simulink model "FMS"  (R2018b)
settings: configuration reference "fms_config" (kept outside this file)
values from neighbouring files (symbols this model uses):
  FMS_EXPORT = Simulink.Parameter(FMS_EXPORT_VALUE)    [fms_model_init.m]
  FMS_PARAM = Simulink.Parameter(FMS_PARAM_VALUE)    [fms_model_init.m]
undefined symbols (not defined in the file or in its folder): actuator_cmd, ax_cmd, ay_cmd, az_cmd, cmd_mask, ControlMode, ctrl_mode, DiscIntNeverNeededParam, ext_state, FMS_Cmd, FMS_CONST, home, mode, p_cmd, phi_cmd, PilotMode, psi_rate_cmd, q_cmd, r_cmd, reset, state, status, theta_cmd, throttle_cmd, timestamp, u_cmd, v_cmd, VehicleState, VehicleStatus, VTOLState, w_cmd, wp_consume, wp_current
libraries: simulink x141, FMT_Model_Lib x120, hdlsllib x13
(part 3 of 12)

== system FMS/FMS Commander/Commander/Arm/MC_Mode/SubMode/Takeoff ==
  FMS_In : Inport
  Action Port : ActionPort  InitializeStates=reset  ActionType=case
      settings: CopyFcn=Stateflow.SLINSF.SimulinkMan.removeBlockPreDeleteFcn
  Bus Assignment1 : BusAssignment  AssignedSignals=status,state,ctrl_mode,psi_rate_cmd,u_cmd,v_cmd,w_cmd
  Climb Speed : Subsystem
  Constant : Constant  Value=0  OutDataTypeStr=Inherit: Inherit via back propagation
  Constant1 : Constant  Value=0  OutDataTypeStr=Bus: FMS_Out_Bus
  Constant2 : Constant  Value=ControlMode.POSCTL
  Constant3 : Constant  Value=VehicleState.Takeoff
  Constant5 : Constant  Value=VehicleStatus.Arm
  Data Type Conversion : DataTypeConversion
  Data Type Conversion1 : DataTypeConversion
  Data Type Conversion2 : DataTypeConversion
  Demux : Demux  Outputs=2
  Track Position : Subsystem
  FMS_Out : Outport
  wires:
  Constant5/1 -> Data Type Conversion/1
  Demux/2 -> Bus Assignment1/7
  Demux/1 -> Bus Assignment1/6
  Constant/1 -> Bus Assignment1/5
  Constant2/1 -> Data Type Conversion2/1
  Track Position/1(uv_cmd_mPs) -> Demux/1
  Constant1/1 -> Bus Assignment1/1
  FMS_In/1 -> Climb Speed/1(FMS_In), Track Position/1(FMS_In)
  Bus Assignment1/1 -> FMS_Out/1
  Data Type Conversion/1 -> Bus Assignment1/2
  Data Type Conversion1/1 -> Bus Assignment1/3
  Constant3/1 -> Data Type Conversion1/1
  Data Type Conversion2/1 -> Bus Assignment1/4
  Climb Speed/1(w_cmd_mPs) -> Bus Assignment1/8

== system FMS/FMS Commander/Commander/Arm/MC_Mode/SubMode/Unknown ==
  Action Port : ActionPort  InitializeStates=reset  ActionType=default
  Bus Assignment : BusAssignment  AssignedSignals=reset,status,state,actuator_cmd
  Constant : Constant  Value=0  OutDataTypeStr=Bus: FMS_Out_Bus
  Constant1 : Constant  Value=VehicleStatus.Disarm
  Constant2 : Constant  OutDataTypeStr=Inherit: Inherit via back propagation
  Constant3 : Constant  Value=[1000;1000;1000;1000]  VectorParams1D=off  OutDataTypeStr=Inherit: Inherit via back propagation
  Constant4 : Constant  Value=zeros(12,1)  OutDataTypeStr=Inherit: Inherit via back propagation
  Constant5 : Constant  Value=VehicleState.Disarm
  Data Type Conversion : DataTypeConversion
  Data Type Conversion1 : DataTypeConversion
  Mux : Mux  Inputs=2
  FMS_Out : Outport
  wires:
  Mux/1 -> Bus Assignment/5
  Constant4/1 -> Mux/2
  Constant3/1 -> Mux/1
  Constant1/1 -> Data Type Conversion/1
  Constant2/1 -> Bus Assignment/2
  Bus Assignment/1 -> FMS_Out/1
  Constant/1 -> Bus Assignment/1
  Constant5/1 -> Data Type Conversion1/1
  Data Type Conversion/1 -> Bus Assignment/3
  Data Type Conversion1/1 -> Bus Assignment/4

== system FMS/FMS Commander/Commander/Arm/BackwardTrans_Mode/Position Command/Controller/Brake Control ==
  Action Port : ActionPort  InitializeStates=reset  ActionType=case
  Brake Speed : Constant  Value=0  VectorParams1D=off  OutDataTypeStr=single
  ay_cmd_mPs2 : Outport
  wires:
  Brake Speed/1 -> ay_cmd_mPs2/1

== system FMS/FMS Commander/Commander/Arm/BackwardTrans_Mode/Position Command/Controller/Hold Control ==
  note: Use L1 only if vehicle fly forward
  FMS_In : Inport
  Action Port : ActionPort  InitializeStates=reset  ActionType=case
  Bus Selector1 : BusSelector  OutputSignals=INS_Out.vn,INS_Out.ve
  FMS_In1 : InportShadow
  Fly_Direction : Subsystem
  L1 : Constant  Value=FMS_PARAM.FW_L1  OutDataTypeStr=single
  L1_Reference_WP : Subsystem
  Lateral_Acceleration : Subsystem
  Mux : Mux  Inputs=2
  Path_Ray : Subsystem
  Switch : Switch  Criteria=u2 > Threshold
  Velocity_Controller : Subsystem
  ay_cmd_mPs2 : Outport
  wires:
  FMS_In/1 -> Path_Ray/1(FMS_In)
  Path_Ray/1(p_vehicle) -> Lateral_Acceleration/1(p_vehicle), L1_Reference_WP/1(c)
  Path_Ray/2(p_0) -> L1_Reference_WP/2(p_0)
  Path_Ray/3(n) -> L1_Reference_WP/3(n)
  L1/1 -> L1_Reference_WP/4(L1), Lateral_Acceleration/3(L1)
  FMS_In1/1 -> Fly_Direction/1(FMS_In), Velocity_Controller/1(FMS_In), Bus Selector1/1
  Bus Selector1/1 -> Mux/1  "<vn>"
  Bus Selector1/2 -> Mux/2  "<ve>"
  L1_Reference_WP/1(L1_WP) -> Lateral_Acceleration/2(L1_WP)
  Mux/1 -> Lateral_Acceleration/4(Vg)
  Lateral_Acceleration/1(ay_cmd_mPs2) -> Switch/1
  Fly_Direction/1(sign) -> Switch/2
  Velocity_Controller/1(ay_cmd_B_rad) -> Switch/3
  Switch/1 -> ay_cmd_mPs2/1

== system FMS/FMS Commander/Commander/Arm/BackwardTrans_Mode/Position Command/Controller/Move Control ==
  FMS_In : Inport
  Action Port : ActionPort  InitializeStates=reset  ActionType=case
  Bus Selector : BusSelector  OutputSignals=Pilot_Cmd.stick_roll
  DeadZone1 : Subsystem  mask{th=FMS_PARAM.ROLL_DZ}
      mask prompts: th "Threshold"
      mask Display: disp('Dead Zone')
  Gain6 : Gain  Gain=FMS_PARAM.FW_ACC_Y_LIM/2  OutDataTypeStr=single
  TD : Subsystem  Commented=on
  ay_cmd_mPs2 : Outport
  wires:
  DeadZone1/1(y) -> Gain6/1
  Bus Selector/1 -> DeadZone1/1(u)  "<stick_roll>"
  FMS_In/1 -> Bus Selector/1
  Gain6/1 -> ay_cmd_mPs2/1

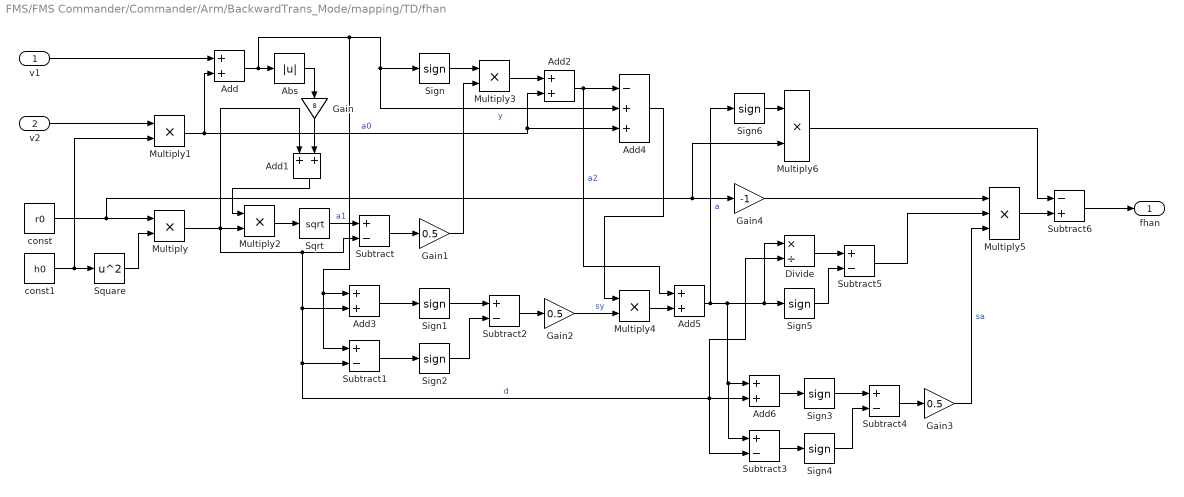
== system FMS/FMS Commander/Commander/Arm/BackwardTrans_Mode/mapping/TD/fhan  ==
  v1 : Inport
  v2 : Inport  Port=2
  Abs : Abs
  Add{,1..3,5..6} (6 alike) : Sum  OutDataTypeStr=Inherit: Same as first input
  Add4 : Sum  Inputs=-++
  Divide : Product  Inputs=*/
  Gain : Gain  Gain=8
  Gain1 : Gain  Gain=0.5  OutDataTypeStr=Inherit: Same as input
  Gain2 : Gain  Gain=0.5  OutDataTypeStr=Inherit: Same as input
  Gain3 : Gain  Gain=0.5  OutDataTypeStr=Inherit: Same as input
  Gain4 : Gain  Gain=-1  OutDataTypeStr=Inherit: Same as input
  Multiply{,1..3} (4 alike) : Product  OutDataTypeStr=Inherit: Same as first input
  Multiply4 : Product  OutDataTypeStr=single
  Multiply5 : Product  Inputs=3
  Multiply6 : Product  OutDataTypeStr=single
  Sign{,1..6} (7 alike) : Signum
  Sqrt : Sqrt  SaturateOnIntegerOverflow=on
  Square : Math  Operator=square  SaturateOnIntegerOverflow=on
  Subtract{,1..5} (6 alike) : Sum  Inputs=+-  OutDataTypeStr=Inherit: Same as first input
  Subtract6 : Sum  Inputs=-+  OutDataTypeStr=Inherit: Same as first input
  const : Constant  Value=r0  OutDataTypeStr=single
  const1 : Constant  Value=h0  OutDataTypeStr=single
  fhan : Outport
  wires:
  v1/1 -> Add/1
  Sign/1 -> Multiply3/1
  Gain2/1 -> Multiply4/2  "sy"
  v2/1 -> Multiply1/1
  Gain3/1 -> Multiply5/3  "sa"
  Subtract/1 -> Gain1/1
  Subtract6/1 -> fhan/1
  Sign2/1 -> Subtract2/2
  Sign4/1 -> Subtract4/2
  Abs/1 -> Gain/1
  Add4/1 -> Multiply4/1
  Sign5/1 -> Subtract5/2
  Sqrt/1 -> Subtract/1  "a1"
  Subtract3/1 -> Sign4/1
  Add1/1 -> Multiply2/1
  Subtract1/1 -> Sign2/1
  Divide/1 -> Subtract5/1
  Multiply3/1 -> Add2/1
  Gain/1 -> Add1/2
  const/1 -> Multiply6/2, Gain4/1, Multiply/1
  Add3/1 -> Sign1/1
  Subtract5/1 -> Multiply5/2
  Multiply4/1 -> Add5/2
  const1/1 -> Multiply1/2, Square/1
  Add5/1 -> Sign6/1, Sign5/1, Divide/1, Subtract3/1, Add6/1  "a"
  Multiply1/1 -> Add4/3, Add2/2, Add/2  "a0"
  Add/1 -> Subtract1/1, Add3/1, Add4/2, Sign/1, Abs/1  "y"
  Subtract2/1 -> Gain2/1
  Add2/1 -> Add4/1, Add5/1  "a2"
  Subtract4/1 -> Gain3/1
  Gain4/1 -> Multiply5/1
  Multiply5/1 -> Subtract6/2
  Sign6/1 -> Multiply6/1
  Sign3/1 -> Subtract4/1
  Add6/1 -> Sign3/1
  Multiply/1 -> Subtract/2, Divide/2, Subtract3/2, Add6/2, Subtract1/2, Add3/2, Add1/1, Multiply2/2  "d"
  Multiply6/1 -> Subtract6/1
  Gain1/1 -> Multiply3/2
  Square/1 -> Multiply/2
  Multiply2/1 -> Sqrt/1
  Sign1/1 -> Subtract2/1

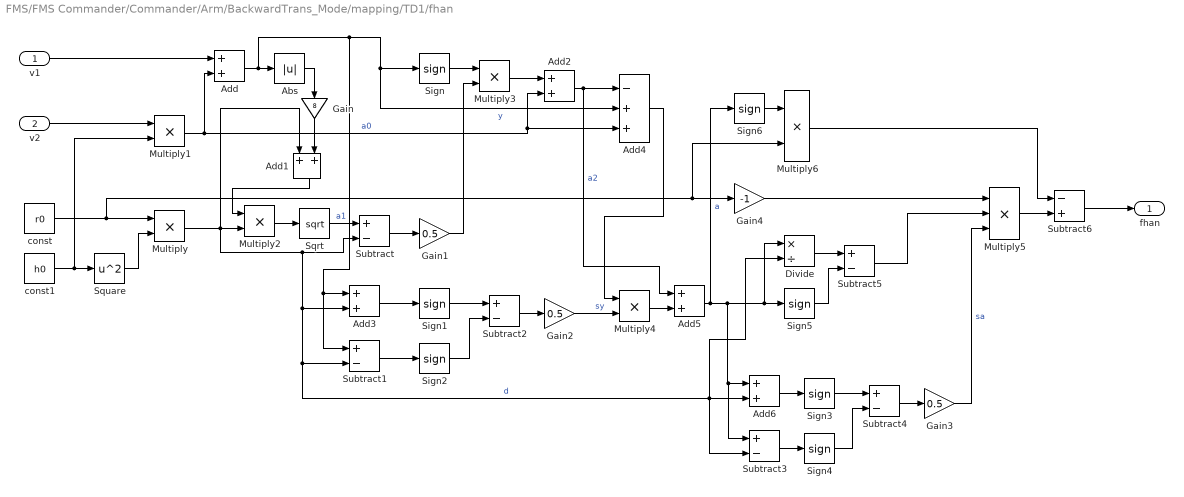
== system FMS/FMS Commander/Commander/Arm/BackwardTrans_Mode/mapping/TD1/fhan  ==
  v1 : Inport
  v2 : Inport  Port=2
  Abs : Abs
  Add{,1..3,5..6} (6 alike) : Sum  OutDataTypeStr=Inherit: Same as first input
  Add4 : Sum  Inputs=-++
  Divide : Product  Inputs=*/
  Gain : Gain  Gain=8
  Gain1 : Gain  Gain=0.5  OutDataTypeStr=Inherit: Same as input
  Gain2 : Gain  Gain=0.5  OutDataTypeStr=Inherit: Same as input
  Gain3 : Gain  Gain=0.5  OutDataTypeStr=Inherit: Same as input
  Gain4 : Gain  Gain=-1  OutDataTypeStr=Inherit: Same as input
  Multiply{,1..3} (4 alike) : Product  OutDataTypeStr=Inherit: Same as first input
  Multiply4 : Product  OutDataTypeStr=single
  Multiply5 : Product  Inputs=3
  Multiply6 : Product  OutDataTypeStr=single
  Sign{,1..6} (7 alike) : Signum
  Sqrt : Sqrt  SaturateOnIntegerOverflow=on
  Square : Math  Operator=square  SaturateOnIntegerOverflow=on
  Subtract{,1..5} (6 alike) : Sum  Inputs=+-  OutDataTypeStr=Inherit: Same as first input
  Subtract6 : Sum  Inputs=-+  OutDataTypeStr=Inherit: Same as first input
  const : Constant  Value=r0  OutDataTypeStr=single
  const1 : Constant  Value=h0  OutDataTypeStr=single
  fhan : Outport
  wires:
  v1/1 -> Add/1
  Sign/1 -> Multiply3/1
  Gain2/1 -> Multiply4/2  "sy"
  v2/1 -> Multiply1/1
  Gain3/1 -> Multiply5/3  "sa"
  Subtract/1 -> Gain1/1
  Subtract6/1 -> fhan/1
  Sign2/1 -> Subtract2/2
  Sign4/1 -> Subtract4/2
  Abs/1 -> Gain/1
  Add4/1 -> Multiply4/1
  Sign5/1 -> Subtract5/2
  Sqrt/1 -> Subtract/1  "a1"
  Subtract3/1 -> Sign4/1
  Add1/1 -> Multiply2/1
  Subtract1/1 -> Sign2/1
  Divide/1 -> Subtract5/1
  Multiply3/1 -> Add2/1
  Gain/1 -> Add1/2
  const/1 -> Multiply6/2, Gain4/1, Multiply/1
  Add3/1 -> Sign1/1
  Subtract5/1 -> Multiply5/2
  Multiply4/1 -> Add5/2
  const1/1 -> Multiply1/2, Square/1
  Add5/1 -> Sign6/1, Sign5/1, Divide/1, Subtract3/1, Add6/1  "a"
  Multiply1/1 -> Add4/3, Add2/2, Add/2  "a0"
  Add/1 -> Subtract1/1, Add3/1, Add4/2, Sign/1, Abs/1  "y"
  Subtract2/1 -> Gain2/1
  Add2/1 -> Add4/1, Add5/1  "a2"
  Subtract4/1 -> Gain3/1
  Gain4/1 -> Multiply5/1
  Multiply5/1 -> Subtract6/2
  Sign6/1 -> Multiply6/1
  Sign3/1 -> Subtract4/1
  Add6/1 -> Sign3/1
  Multiply/1 -> Subtract/2, Divide/2, Subtract3/2, Add6/2, Subtract1/2, Add3/2, Add1/1, Multiply2/2  "d"
  Multiply6/1 -> Subtract6/1
  Gain1/1 -> Multiply3/2
  Square/1 -> Multiply/2
  Multiply2/1 -> Sqrt/1
  Sign1/1 -> Subtract2/1

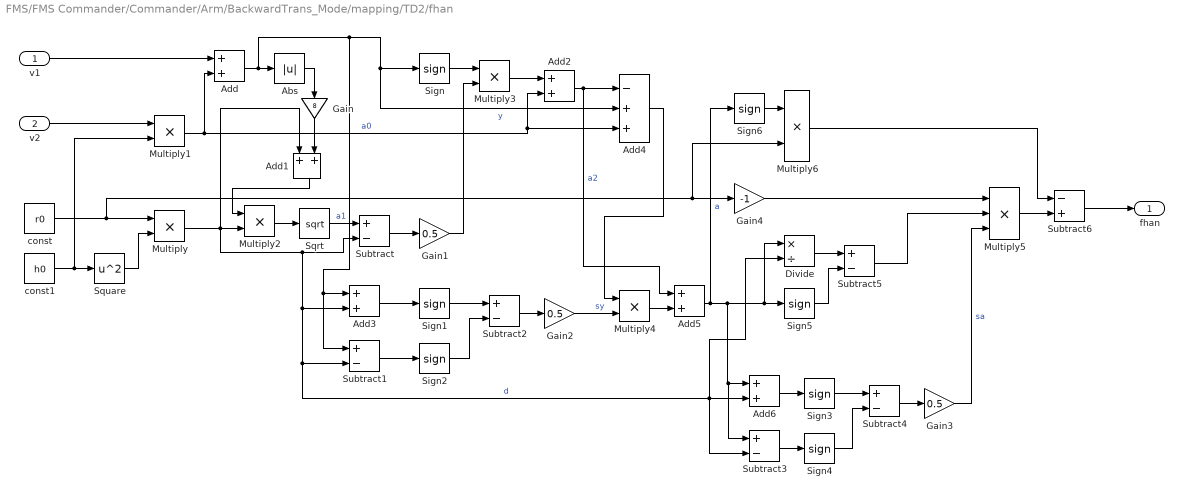
== system FMS/FMS Commander/Commander/Arm/BackwardTrans_Mode/mapping/TD2/fhan  ==
  v1 : Inport
  v2 : Inport  Port=2
  Abs : Abs
  Add{,1..3,5..6} (6 alike) : Sum  OutDataTypeStr=Inherit: Same as first input
  Add4 : Sum  Inputs=-++
  Divide : Product  Inputs=*/
  Gain : Gain  Gain=8
  Gain1 : Gain  Gain=0.5  OutDataTypeStr=Inherit: Same as input
  Gain2 : Gain  Gain=0.5  OutDataTypeStr=Inherit: Same as input
  Gain3 : Gain  Gain=0.5  OutDataTypeStr=Inherit: Same as input
  Gain4 : Gain  Gain=-1  OutDataTypeStr=Inherit: Same as input
  Multiply{,1..3} (4 alike) : Product  OutDataTypeStr=Inherit: Same as first input
  Multiply4 : Product  OutDataTypeStr=single
  Multiply5 : Product  Inputs=3
  Multiply6 : Product  OutDataTypeStr=single
  Sign{,1..6} (7 alike) : Signum
  Sqrt : Sqrt  SaturateOnIntegerOverflow=on
  Square : Math  Operator=square  SaturateOnIntegerOverflow=on
  Subtract{,1..5} (6 alike) : Sum  Inputs=+-  OutDataTypeStr=Inherit: Same as first input
  Subtract6 : Sum  Inputs=-+  OutDataTypeStr=Inherit: Same as first input
  const : Constant  Value=r0  OutDataTypeStr=single
  const1 : Constant  Value=h0  OutDataTypeStr=single
  fhan : Outport
  wires:
  Sign1/1 -> Subtract2/1
  Multiply2/1 -> Sqrt/1
  Square/1 -> Multiply/2
  Gain1/1 -> Multiply3/2
  Multiply6/1 -> Subtract6/1
  Multiply/1 -> Multiply2/2, Add1/1, Add3/2, Subtract1/2, Add6/2, Subtract3/2, Divide/2, Subtract/2  "d"
  Add6/1 -> Sign3/1
  Sign3/1 -> Subtract4/1
  Sign6/1 -> Multiply6/1
  Multiply5/1 -> Subtract6/2
  Gain4/1 -> Multiply5/1
  Subtract4/1 -> Gain3/1
  Add2/1 -> Add5/1, Add4/1  "a2"
  Subtract2/1 -> Gain2/1
  Add/1 -> Abs/1, Sign/1, Add4/2, Add3/1, Subtract1/1  "y"
  Multiply1/1 -> Add/2, Add2/2, Add4/3  "a0"
  Add5/1 -> Add6/1, Subtract3/1, Divide/1, Sign5/1, Sign6/1  "a"
  const1/1 -> Square/1, Multiply1/2
  Multiply4/1 -> Add5/2
  Subtract5/1 -> Multiply5/2
  Add3/1 -> Sign1/1
  const/1 -> Multiply/1, Gain4/1, Multiply6/2
  Gain/1 -> Add1/2
  Multiply3/1 -> Add2/1
  Divide/1 -> Subtract5/1
  Subtract1/1 -> Sign2/1
  Add1/1 -> Multiply2/1
  Subtract3/1 -> Sign4/1
  Sqrt/1 -> Subtract/1  "a1"
  Sign5/1 -> Subtract5/2
  Add4/1 -> Multiply4/1
  Abs/1 -> Gain/1
  Sign4/1 -> Subtract4/2
  Sign2/1 -> Subtract2/2
  Subtract6/1 -> fhan/1
  Subtract/1 -> Gain1/1
  Gain3/1 -> Multiply5/3  "sa"
  v2/1 -> Multiply1/1
  Gain2/1 -> Multiply4/2  "sy"
  Sign/1 -> Multiply3/1
  v1/1 -> Add/1

== system FMS/FMS Commander/Commander/Arm/FW_Mode/Assist/Altitude/Altitude Command ==
  FMS_In : Inport
  Controller : Subsystem
  Detect Movement : Subsystem
  w_cmd_mPs : Outport
  wires:
  Controller/1(w_cmd_mPs) -> w_cmd_mPs/1
  Detect Movement/1(motion_state) -> Controller/1(motion_state)
  FMS_In/1 -> Controller/2(FMS_In), Detect Movement/1(FMS_In)

== system FMS/FMS Commander/Commander/Arm/FW_Mode/Assist/Altitude/Attitude Command ==
  FMS_In : Inport
  Bus Selector : BusSelector  OutputSignals=Pilot_Cmd.stick_roll
  DeadZone : Subsystem  mask{th=FMS_PARAM.ROLL_DZ}
      mask prompts: th "Threshold"
      mask Display: disp('Dead Zone')
  Gain : Gain  Gain=FMS_PARAM.FW_ROLL_LIM
  TD : Subsystem
  phi_cmd_radPs : Outport
  wires:
  Bus Selector/1 -> DeadZone/1(u)  "<stick_roll>"
  FMS_In/1 -> Bus Selector/1
  DeadZone/1(y) -> Gain/1
  Gain/1 -> TD/1(v)
  TD/1(v1) -> phi_cmd_radPs/1

== system FMS/FMS Commander/Commander/Arm/FW_Mode/Assist/Altitude/Heading Command ==
  FMS_In : Inport
  Bus Selector : BusSelector  OutputSignals=Pilot_Cmd.stick_yaw
  DeadZone : Subsystem  mask{th=FMS_PARAM.YAW_DZ}
      mask prompts: th "Threshold"
      mask Display: disp('Dead Zone')
  Gain1 : Gain  Gain=FMS_PARAM.FW_YAW_RATE_LIM  OutDataTypeStr=single
  TD : Subsystem
  psi_rate_cmd_radPs : Outport
  wires:
  Gain1/1 -> TD/1(v)
  FMS_In/1 -> Bus Selector/1
  DeadZone/1(y) -> Gain1/1
  Bus Selector/1 -> DeadZone/1(u)  "<stick_yaw>"
  TD/1(v1) -> psi_rate_cmd_radPs/1

== system FMS/FMS Commander/Commander/Arm/FW_Mode/Assist/Altitude/Speed Command ==
  FMS_In : Inport
  Bus Selector : BusSelector  OutputSignals=Pilot_Cmd.stick_throttle
  Saturation : Saturate  UpperLimit=1  LowerLimit=-1
  Saturation1 : Saturate  UpperLimit=FMS_PARAM.FW_SPEED_MAX  LowerLimit=FMS_PARAM.FW_SPEED_MIN
  StickToVelMapping : Subsystem  mask{min=FMS_PARAM.FW_SPEED_MIN, mid=FMS_PARAM.FW_CRUISE_SPEED, max=FMS_PARAM.FW_SPEED_MAX}
  TD : Subsystem
  u_cmd_mPs : Outport
  wires:
  FMS_In/1 -> Bus Selector/1
  Bus Selector/1 -> Saturation/1  "<stick_throttle>"
  Saturation/1 -> StickToVelMapping/1(In)
  StickToVelMapping/1(Out) -> TD/1(v)
  Saturation1/1 -> u_cmd_mPs/1
  TD/1(v1) -> Saturation1/1

== system FMS/FMS Commander/Commander/Arm/FW_Mode/Assist/Position/Altitude Command ==
  FMS_In : Inport
  Controller : Subsystem
  Detect Movement : Subsystem
  w_cmd_mPs : Outport
  wires:
  Controller/1(w_cmd_mPs) -> w_cmd_mPs/1
  Detect Movement/1(motion_state) -> Controller/1(motion_state)
  FMS_In/1 -> Controller/2(FMS_In), Detect Movement/1(FMS_In)

== system FMS/FMS Commander/Commander/Arm/FW_Mode/Assist/Position/Heading Command ==
  FMS_In : Inport
  Bus Selector : BusSelector  OutputSignals=Pilot_Cmd.stick_yaw
  DeadZone : Subsystem  mask{th=FMS_PARAM.YAW_DZ}
      mask prompts: th "Threshold"
      mask Display: disp('Dead Zone')
  Gain1 : Gain  Gain=FMS_PARAM.FW_YAW_RATE_LIM  OutDataTypeStr=single
  TD : Subsystem
  psi_rate_cmd_radPs : Outport
  wires:
  Gain1/1 -> TD/1(v)
  FMS_In/1 -> Bus Selector/1
  DeadZone/1(y) -> Gain1/1
  Bus Selector/1 -> DeadZone/1(u)  "<stick_yaw>"
  TD/1(v1) -> psi_rate_cmd_radPs/1

== system FMS/FMS Commander/Commander/Arm/FW_Mode/Assist/Position/Position Command ==
  FMS_In : Inport
  Controller : Subsystem
  Detect Movement : Subsystem
  ay_cmd_mPs2 : Outport
  wires:
  FMS_In/1 -> Controller/2(FMS_In), Detect Movement/1(FMS_In)
  Controller/1(ay_cmd_mPs2) -> ay_cmd_mPs2/1
  Detect Movement/1(motion_state) -> Controller/1(motion_state)

== system FMS/FMS Commander/Commander/Arm/FW_Mode/Assist/Position/Speed Command ==
  FMS_In : Inport
  Bus Selector : BusSelector  OutputSignals=Pilot_Cmd.stick_throttle
  Saturation : Saturate  UpperLimit=1  LowerLimit=-1
  Saturation1 : Saturate  UpperLimit=FMS_PARAM.FW_SPEED_MAX  LowerLimit=FMS_PARAM.FW_SPEED_MIN
  StickToVelMapping : Subsystem  mask{min=FMS_PARAM.FW_SPEED_MIN, mid=FMS_PARAM.FW_CRUISE_SPEED, max=FMS_PARAM.FW_SPEED_MAX}
  TD : Subsystem
  u_cmd_mPs : Outport
  wires:
  FMS_In/1 -> Bus Selector/1
  Bus Selector/1 -> Saturation/1  "<stick_throttle>"
  Saturation/1 -> StickToVelMapping/1(In)
  StickToVelMapping/1(Out) -> TD/1(v)
  Saturation1/1 -> u_cmd_mPs/1
  TD/1(v1) -> Saturation1/1

== system FMS/FMS Commander/Commander/Arm/FW_Mode/Assist/Stabilize/Attitude Command ==
  FMS_In : Inport
  Bus Selector : BusSelector  OutputSignals=Pilot_Cmd.stick_roll,Pilot_Cmd.stick_pitch
  DeadZone : Subsystem  mask{th=FMS_PARAM.ROLL_DZ}
      mask prompts: th "Threshold"
      mask Display: disp('Dead Zone')
  DeadZone2 : Subsystem  mask{th=FMS_PARAM.PITCH_DZ}
      mask prompts: th "Threshold"
      mask Display: disp('Dead Zone')
  Gain : Gain  Gain=FMS_PARAM.FW_ROLL_LIM
  Gain1 : Gain  Gain=-FMS_PARAM.FW_PITCH_LIM
  Phi_CMD_TD : Subsystem
  Theta_CMD_TD : Subsystem
  phi_cmd_radPs : Outport
  theta_cmd_radPs : Outport  Port=2
  wires:
  Bus Selector/2 -> DeadZone2/1(u)  "<stick_pitch>"
  Bus Selector/1 -> DeadZone/1(u)  "<stick_roll>"
  FMS_In/1 -> Bus Selector/1
  DeadZone2/1(y) -> Gain1/1
  DeadZone/1(y) -> Gain/1
  Gain/1 -> Phi_CMD_TD/1(v)
  Gain1/1 -> Theta_CMD_TD/1(v)
  Phi_CMD_TD/1(v1) -> phi_cmd_radPs/1
  Theta_CMD_TD/1(v1) -> theta_cmd_radPs/1

== system FMS/FMS Commander/Commander/Arm/FW_Mode/Assist/Stabilize/Heading Command ==
  FMS_In : Inport
  Bus Selector : BusSelector  OutputSignals=Pilot_Cmd.stick_yaw
  DeadZone : Subsystem  mask{th=FMS_PARAM.YAW_DZ}
      mask prompts: th "Threshold"
      mask Display: disp('Dead Zone')
  Gain1 : Gain  Gain=FMS_PARAM.FW_YAW_RATE_LIM  OutDataTypeStr=single
  TD : Subsystem
  psi_rate_cmd_radPs : Outport
  wires:
  Gain1/1 -> TD/1(v)
  FMS_In/1 -> Bus Selector/1
  DeadZone/1(y) -> Gain1/1
  Bus Selector/1 -> DeadZone/1(u)  "<stick_yaw>"
  TD/1(v1) -> psi_rate_cmd_radPs/1

== system FMS/FMS Commander/Commander/Arm/FW_Mode/Assist/Stabilize/Throttle Command ==
  FMS_In : Inport
  Add : Sum
  Bus Selector : BusSelector  OutputSignals=Pilot_Cmd.stick_throttle
  Constant5 : Constant  Value=1000  OutDataTypeStr=uint16
  Gain2 : Gain  Gain=1000  OutDataTypeStr=uint16
  Saturation : Saturate  UpperLimit=1  LowerLimit=0
  throttle_cmd : Outport
  wires:
  FMS_In/1 -> Bus Selector/1
  Gain2/1 -> Add/1
  Saturation/1 -> Gain2/1
  Bus Selector/1 -> Saturation/1  "<stick_throttle>"
  Constant5/1 -> Add/2
  Add/1 -> throttle_cmd/1

== system FMS/FMS Commander/Commander/Arm/FW_Mode/Auto/Mission/Mission_SubSystem ==
  FMS_In : Inport
  Reset : ResetPort  DisableCoverage=on
  Altitude Control : Subsystem
  Bus Assignment : BusAssignment  AssignedSignals=status,state,ctrl_mode,u_cmd,ay_cmd,w_cmd
  Constant : Constant  Value=0  OutDataTypeStr=Bus: FMS_Out_Bus
  Constant1 : Constant  Value=VehicleStatus.Arm
  Constant2 : Constant  Value=VehicleState.Mission
  Constant3 : Constant  Value=ControlMode.POSCTL
  Cruise_Speed : Subsystem
  Data Type Conversion : DataTypeConversion
  Data Type Conversion1 : DataTypeConversion
  Data Type Conversion2 : DataTypeConversion
  Position Command : Subsystem
  FMS_Out : Outport
  wires:
  Data Type Conversion1/1 -> Bus Assignment/3
  Constant1/1 -> Data Type Conversion/1
  Data Type Conversion2/1 -> Bus Assignment/4
  Data Type Conversion/1 -> Bus Assignment/2
  Constant2/1 -> Data Type Conversion1/1
  Constant3/1 -> Data Type Conversion2/1
  Constant/1 -> Bus Assignment/1
  Bus Assignment/1 -> FMS_Out/1
  FMS_In/1 -> Cruise_Speed/1(FMS_In), Altitude Control/1(FMS_In), Position Command/1(FMS_In)
  Position Command/1(ay_cmd_mPs2) -> Bus Assignment/6
  Altitude Control/1(w_cmd_mPs) -> Bus Assignment/7
  Cruise_Speed/1(u_cmd) -> Bus Assignment/5

== system FMS/FMS Commander/Commander/Arm/FW_Mode/SubMode/Hold/Altitude_Hold ==
  FMS_In : Inport
  Bus_Selection : Subsystem
  Delay : Delay  DelayLength=1  InitialConditionSource=Input port
      settings: InputPortMap=u0,p4
  Gain2 : Gain  Gain=FMS_PARAM.Z_P  OutDataTypeStr=single
  Saturation1 : Saturate  UpperLimit=FMS_PARAM.VEL_Z_LIM  LowerLimit=-FMS_PARAM.VEL_Z_LIM
  Sum : Sum  Inputs=-+|
  w_cmd_mPs : Outport
  wires:
  Gain2/1 -> Saturation1/1
  Bus_Selection/1(z_R_m) -> Delay/2, Sum/1  "z_est_R"
  Sum/1 -> Gain2/1  "z_err_R"
  Delay/1 -> Sum/2, Delay/1  "z_cmd_R"
  FMS_In/1 -> Bus_Selection/1(FMS_In)
  Saturation1/1 -> w_cmd_mPs/1

== system FMS/FMS Commander/Commander/Arm/FW_Mode/SubMode/Hold/Loiter_Control ==
  FMS_In : Inport
  Bus Selector2 : BusSelector  OutputSignals=INS_Out.vn,INS_Out.ve
  L1 : Constant  Value=FMS_PARAM.FW_L1  OutDataTypeStr=single
  L1 Reference WP : Subsystem
  L1_Core : Subsystem
  Mux1 : Mux  Inputs=2
  R : Constant  Value=FMS_PARAM.FW_LOITER_R  OutDataTypeStr=single
  Reference_Point : Subsystem
  Saturation1 : Saturate  UpperLimit=FMS_PARAM.FW_ACC_Y_LIM  LowerLimit=-FMS_PARAM.FW_ACC_Y_LIM
  ay_cmd_mPs2 : Outport
  wires:
  L1 Reference WP/1(L1_WP) -> L1_Core/2(L1_WP)  "L1_WP"
  L1_Core/1(ay_cmd_mPs2) -> Saturation1/1
  Reference_Point/1(p_vehicle) -> L1_Core/1(p_vehicle), L1 Reference WP/1(P_Vehicle)
  Reference_Point/2(p_0) -> L1 Reference WP/2(P_0)
  Reference_Point/3(n) -> L1 Reference WP/3(n)
  R/1 -> L1 Reference WP/4(R)
  L1/1 -> L1_Core/3(L1), L1 Reference WP/5(L1)
  FMS_In/1 -> Bus Selector2/1, Reference_Point/1(FMS_In)
  Bus Selector2/2 -> Mux1/2  "<ve>"
  Bus Selector2/1 -> Mux1/1  "<vn>"
  Mux1/1 -> L1_Core/4(Vg)
  Saturation1/1 -> ay_cmd_mPs2/1

== system FMS/FMS Commander/Commander/Arm/FW_Mode/SubMode/Return/Altitude Control ==
  FMS_In : Inport
  Bus Selector3 : BusSelector  OutputSignals=INS_Out.h_R
  Gain : Gain  Gain=FMS_PARAM.FW_Z_P
  Saturation1 : Saturate  UpperLimit=FMS_PARAM.FW_VEL_Z_LIM  LowerLimit=-FMS_PARAM.FW_VEL_Z_LIM
  Sum2 : Sum  Inputs=|+-
  Target Height : Subsystem
  w_cmd_mPs : Outport
  wires:
  FMS_In/1 -> Bus Selector3/1, Target Height/1(FMS_In)
  Bus Selector3/1 -> Sum2/1  "<h_R>"
  Sum2/1 -> Gain/1
  Gain/1 -> Saturation1/1
  Target Height/1(h_R_sp) -> Sum2/2  "h_R_sp"
  Saturation1/1 -> w_cmd_mPs/1

== system FMS/FMS Commander/Commander/Arm/FW_Mode/SubMode/Return/Position Command ==
  FMS_In : Inport
  L1 Control : Subsystem
  WayPoints : Subsystem
  ay_cmd_mPs2 : Outport
  wires:
  FMS_In/1 -> L1 Control/4(FMS_In), WayPoints/1(FMS_In)
  L1 Control/1(ay_cmd_mPs2) -> ay_cmd_mPs2/1
  WayPoints/2(p2) -> L1 Control/2(p2)
  WayPoints/3(p3) -> L1 Control/3(p3)
  WayPoints/1(p1) -> L1 Control/1(p1)

== system FMS/FMS Commander/Commander/Arm/FW_Mode/SubMode/Takeoff/Altitude Control ==
  FMS_In : Inport
  Bus Selector3 : BusSelector  OutputSignals=INS_Out.h_R
  Gain : Gain  Gain=FMS_PARAM.FW_Z_P
  Saturation1 : Saturate  UpperLimit=FMS_PARAM.FW_VEL_Z_LIM  LowerLimit=-FMS_PARAM.FW_VEL_Z_LIM
  Sum2 : Sum  Inputs=|+-
  Target Height : Subsystem
  w_cmd_mPs : Outport
  wires:
  FMS_In/1 -> Bus Selector3/1, Target Height/1(FMS_In)
  Bus Selector3/1 -> Sum2/1  "<h_R>"
  Sum2/1 -> Gain/1
  Gain/1 -> Saturation1/1
  Target Height/1(h_R_sp) -> Sum2/2  "h_R_sp"
  Saturation1/1 -> w_cmd_mPs/1

== system FMS/FMS Commander/Commander/Arm/FW_Mode/SubMode/Takeoff/Position Command ==
  FMS_In : Inport
  L1 Control : Subsystem
  WayPoints : Subsystem
  ay_cmd_mPs2 : Outport
  wires:
  FMS_In/1 -> L1 Control/4(FMS_In), WayPoints/1(FMS_In)
  L1 Control/1(ay_cmd_mPs2) -> ay_cmd_mPs2/1
  WayPoints/2(p2) -> L1 Control/2(p2)
  WayPoints/3(p3) -> L1 Control/3(p3)
  WayPoints/1(p1) -> L1 Control/1(p1)

== system FMS/FMS Commander/Commander/Arm/MC_Mode/Assist/Acro/Angular Rate Command ==
  FMS_In : Inport
  Bus Selector : BusSelector  OutputSignals=Pilot_Cmd.stick_roll,Pilot_Cmd.stick_pitch,Pilot_Cmd.stick_yaw
  Gain : Gain  Gain=pi  OutDataTypeStr=single
  Gain1 : Gain  Gain=-pi  OutDataTypeStr=single
  Gain2 : Gain  Gain=pi/2  OutDataTypeStr=single
  p_cmd_radPs : Outport
  q_cmd_radPs : Outport  Port=2
  r_cmd_radPs : Outport  Port=3
  wires:
  FMS_In/1 -> Bus Selector/1
  Gain2/1 -> r_cmd_radPs/1
  Gain1/1 -> q_cmd_radPs/1
  Bus Selector/3 -> Gain2/1  "<stick_yaw>"
  Bus Selector/2 -> Gain1/1  "<stick_pitch>"
  Gain/1 -> p_cmd_radPs/1
  Bus Selector/1 -> Gain/1  "<stick_roll>"

== system FMS/FMS Commander/Commander/Arm/MC_Mode/Assist/Acro/Throttle Command ==
  FMS_In : Inport
  Add : Sum
  Bus Selector : BusSelector  OutputSignals=Pilot_Cmd.stick_throttle
  Constant4 : Constant  OutDataTypeStr=single
  Constant5 : Constant  Value=1000  OutDataTypeStr=uint16
  Gain2 : Gain  Gain=500  OutDataTypeStr=uint16
  Saturation : Saturate  UpperLimit=2  LowerLimit=0
  Sum : Sum  Inputs=|++
  throttle_cmd : Outport
  wires:
  Constant4/1 -> Sum/2
  Add/1 -> throttle_cmd/1
  Constant5/1 -> Add/2
  Bus Selector/1 -> Sum/1  "<stick_throttle>"
  Saturation/1 -> Gain2/1
  Sum/1 -> Saturation/1
  Gain2/1 -> Add/1
  FMS_In/1 -> Bus Selector/1

== system FMS/FMS Commander/Commander/Arm/MC_Mode/Assist/Altitude/Altitude Command ==
  FMS_In : Inport
  Bus Selector : BusSelector  OutputSignals=pilot_cmd_lost
  Constant : Constant  Value=0.5  OutDataTypeStr=single
  Controller : Subsystem
  Detect Movement : Subsystem
  Switch : Switch  Criteria=u2 > Threshold
  w_cmd_mPs : Outport
  wires:
  Controller/1(w_cmd_mPs) -> Switch/3
  Detect Movement/1(motion_state) -> Controller/1(motion_state)
  FMS_In/1 -> Bus Selector/1, Controller/2(FMS_In), Detect Movement/1(FMS_In)
  Bus Selector/1 -> Switch/2  "<pilot_cmd_lost>"
  Constant/1 -> Switch/1
  Switch/1 -> w_cmd_mPs/1

== system FMS/FMS Commander/Commander/Arm/MC_Mode/Assist/Altitude/Attitude Command ==
  FMS_In : Inport
  Bus Selector : BusSelector  OutputSignals=Pilot_Cmd.stick_roll,Pilot_Cmd.stick_pitch
  Bus Selector1 : BusSelector  OutputSignals=pilot_cmd_lost
  Data Type Conversion : DataTypeConversion  OutDataTypeStr=single
  DeadZone : Subsystem  mask{th=FMS_PARAM.ROLL_DZ}
      mask prompts: th "Threshold"
      mask Display: disp('Dead Zone')
  DeadZone2 : Subsystem  mask{th=FMS_PARAM.PITCH_DZ}
      mask prompts: th "Threshold"
      mask Display: disp('Dead Zone')
  Gain : Gain  Gain=FMS_PARAM.ROLL_PITCH_LIM
  Gain1 : Gain  Gain=-FMS_PARAM.ROLL_PITCH_LIM
  Logical Operator : Logic  Operator=NOT  AllPortsSameDT=off  OutDataTypeStr=boolean
  Multiply : Product
  Multiply1 : Product
  Phi_CMD_TD : Subsystem
  Theta_CMD_TD : Subsystem
  phi_cmd_radPs : Outport
  theta_cmd_radPs : Outport  Port=2
  wires:
  Bus Selector/2 -> DeadZone2/1(u)  "<stick_pitch>"
  Bus Selector/1 -> DeadZone/1(u)  "<stick_roll>"
  FMS_In/1 -> Bus Selector1/1, Bus Selector/1
  Phi_CMD_TD/1(v1) -> Multiply/2
  Gain1/1 -> Theta_CMD_TD/1(v)
  Gain/1 -> Phi_CMD_TD/1(v)
  DeadZone2/1(y) -> Gain1/1
  DeadZone/1(y) -> Gain/1
  Bus Selector1/1 -> Logical Operator/1  "<pilot_cmd_lost>"
  Multiply/1 -> phi_cmd_radPs/1
  Theta_CMD_TD/1(v1) -> Multiply1/2
  Multiply1/1 -> theta_cmd_radPs/1
  Logical Operator/1 -> Data Type Conversion/1
  Data Type Conversion/1 -> Multiply1/1, Multiply/1

== system FMS/FMS Commander/Commander/Arm/MC_Mode/Assist/Altitude/Heading Command ==
  FMS_In : Inport
  Controller : Subsystem
  Detect Movement : Subsystem
  psi_rate_cmd_radPs : Outport
  wires:
  Controller/1(psi_rate_cmd_radPs) -> psi_rate_cmd_radPs/1
  Detect Movement/1(motion_state) -> Controller/1(motion_state)
  FMS_In/1 -> Controller/2(FMS_In), Detect Movement/1(FMS_In)

== system FMS/FMS Commander/Commander/Arm/MC_Mode/Assist/Position/Altitude Command ==
  FMS_In : Inport
  Controller : Subsystem
  Detect Movement : Subsystem
  w_cmd_mPs : Outport
  wires:
  Controller/1(w_cmd_mPs) -> w_cmd_mPs/1
  Detect Movement/1(motion_state) -> Controller/1(motion_state)
  FMS_In/1 -> Controller/2(FMS_In), Detect Movement/1(FMS_In)

== system FMS/FMS Commander/Commander/Arm/MC_Mode/Assist/Position/Heading Command ==
  FMS_In : Inport
  Controller : Subsystem
  Detect Movement : Subsystem
  psi_rate_cmd_radPs : Outport
  wires:
  Controller/1(psi_rate_cmd_radPs) -> psi_rate_cmd_radPs/1
  Detect Movement/1(motion_state) -> Controller/1(motion_state)
  FMS_In/1 -> Controller/2(FMS_In), Detect Movement/1(FMS_In)

== system FMS/FMS Commander/Commander/Arm/MC_Mode/Assist/Position/Position Command ==
  FMS_In : Inport
  Controller : Subsystem
  Demux : Demux  Outputs=2
  Detect Movement : Subsystem
  u_cmd_mPs : Outport
  v_cmd_mPs : Outport  Port=2
  wires:
  FMS_In/1 -> Controller/2(FMS_In), Detect Movement/1(FMS_In)
  Demux/2 -> v_cmd_mPs/1
  Demux/1 -> u_cmd_mPs/1
  Controller/1(uv_cmd_mPs) -> Demux/1
  Detect Movement/1(motion_state) -> Controller/1(motion_state)

== system FMS/FMS Commander/Commander/Arm/MC_Mode/Assist/Stabilize/Attitude Command ==
  FMS_In : Inport
  Bus Selector : BusSelector  OutputSignals=Pilot_Cmd.stick_roll,Pilot_Cmd.stick_pitch
  Bus Selector1 : BusSelector  OutputSignals=pilot_cmd_lost
  Data Type Conversion : DataTypeConversion  OutDataTypeStr=single
  DeadZone : Subsystem  mask{th=FMS_PARAM.ROLL_DZ}
      mask prompts: th "Threshold"
      mask Display: disp('Dead Zone')
  DeadZone2 : Subsystem  mask{th=FMS_PARAM.PITCH_DZ}
      mask prompts: th "Threshold"
      mask Display: disp('Dead Zone')
  Gain : Gain  Gain=FMS_PARAM.ROLL_PITCH_LIM
  Gain1 : Gain  Gain=-FMS_PARAM.ROLL_PITCH_LIM
  Logical Operator : Logic  Operator=NOT  AllPortsSameDT=off  OutDataTypeStr=boolean
  Multiply : Product
  Multiply1 : Product
  Phi_CMD_TD : Subsystem
  Theta_CMD_TD : Subsystem
  phi_cmd_radPs : Outport
  theta_cmd_radPs : Outport  Port=2
  wires:
  Bus Selector/2 -> DeadZone2/1(u)  "<stick_pitch>"
  Bus Selector/1 -> DeadZone/1(u)  "<stick_roll>"
  FMS_In/1 -> Bus Selector1/1, Bus Selector/1
  Phi_CMD_TD/1(v1) -> Multiply/2
  Gain1/1 -> Theta_CMD_TD/1(v)
  Gain/1 -> Phi_CMD_TD/1(v)
  DeadZone2/1(y) -> Gain1/1
  DeadZone/1(y) -> Gain/1
  Bus Selector1/1 -> Logical Operator/1  "<pilot_cmd_lost>"
  Multiply/1 -> phi_cmd_radPs/1
  Theta_CMD_TD/1(v1) -> Multiply1/2
  Multiply1/1 -> theta_cmd_radPs/1
  Logical Operator/1 -> Data Type Conversion/1
  Data Type Conversion/1 -> Multiply1/1, Multiply/1

== system FMS/FMS Commander/Commander/Arm/MC_Mode/Assist/Stabilize/Heading Command ==
  FMS_In : Inport
  Controller : Subsystem
  Detect Movement : Subsystem
  psi_rate_cmd_radPs : Outport
  wires:
  FMS_In/1 -> Detect Movement/1(FMS_In), Controller/2(FMS_In)
  Controller/1(psi_rate_cmd_radPs) -> psi_rate_cmd_radPs/1
  Detect Movement/1(motion_state) -> Controller/1(motion_state)

== system FMS/FMS Commander/Commander/Arm/MC_Mode/Assist/Stabilize/Throttle Command ==
  FMS_In : Inport
  Add : Sum
  Bus Selector : BusSelector  OutputSignals=Pilot_Cmd.stick_throttle
  Bus Selector1 : BusSelector  OutputSignals=pilot_cmd_lost
  Constant : Constant  Value=FMS_PARAM.LAND_LOCK_THRO  OutDataTypeStr=uint16
  Constant4 : Constant  OutDataTypeStr=single
  Constant5 : Constant  Value=1000  OutDataTypeStr=uint16
  Gain2 : Gain  Gain=500  OutDataTypeStr=uint16
  Saturation : Saturate  UpperLimit=2  LowerLimit=0
  Sum : Sum  Inputs=|++
  Switch : Switch  Criteria=u2 > Threshold
  throttle_cmd : Outport
  wires:
  FMS_In/1 -> Bus Selector1/1, Bus Selector/1
  Gain2/1 -> Add/1
  Sum/1 -> Saturation/1
  Saturation/1 -> Gain2/1
  Bus Selector/1 -> Sum/1  "<stick_throttle>"
  Constant5/1 -> Add/2
  Add/1 -> Switch/3
  Constant4/1 -> Sum/2
  Bus Selector1/1 -> Switch/2  "<pilot_cmd_lost>"
  Switch/1 -> throttle_cmd/1
  Constant/1 -> Switch/1

== system FMS/FMS Commander/Commander/Arm/MC_Mode/Auto/Mission/Mission_SubSystem ==
  FMS_In : Inport
  Reset : ResetPort  DisableCoverage=on
  Bus Assignment : BusAssignment  AssignedSignals=status,state,ctrl_mode,u_cmd,v_cmd,w_cmd,psi_rate_cmd
  Constant : Constant  Value=0  OutDataTypeStr=Bus: FMS_Out_Bus
  Constant1 : Constant  Value=VehicleStatus.Arm
  Constant2 : Constant  Value=VehicleState.Mission
  Constant3 : Constant  Value=ControlMode.POSCTL
  Data Type Conversion : DataTypeConversion
  Data Type Conversion1 : DataTypeConversion
  Data Type Conversion2 : DataTypeConversion
  Heading Commander : Subsystem
  L1 : Constant  Value=FMS_PARAM.L1  OutDataTypeStr=single
  Sum : Sum  Inputs=+-|
  Velocity Commander : Subsystem
  Way Points : Subsystem
  FMS_Out : Outport
  wires:
  Data Type Conversion1/1 -> Bus Assignment/3
  Way Points/2(p2) -> Velocity Commander/2(p2), Sum/1
  Constant1/1 -> Data Type Conversion/1
  Heading Commander/2(psi_rad_cmd) -> Bus Assignment/8
  L1/1 -> Velocity Commander/4(L1)
  Data Type Conversion2/1 -> Bus Assignment/4
  Data Type Conversion/1 -> Bus Assignment/2
  Constant2/1 -> Data Type Conversion1/1
  Way Points/1(p1) -> Velocity Commander/1(p1), Sum/2
  Way Points/3(p3) -> Velocity Commander/3(p3)
  Velocity Commander/2(v_cmd) -> Bus Assignment/6
  Heading Commander/1(psi_err_rad) -> Velocity Commander/6(psi_err_rad)
  Constant3/1 -> Data Type Conversion2/1
  Constant/1 -> Bus Assignment/1
  Velocity Commander/3(w_cmd) -> Bus Assignment/7
  FMS_In/1 -> Velocity Commander/5(FMS_In), Heading Commander/1(FMS_In), Way Points/1(FMS_In)
  Sum/1 -> Heading Commander/2(p1p2)
  Velocity Commander/1(u_cmd) -> Bus Assignment/5
  Bus Assignment/1 -> FMS_Out/1

== system FMS/FMS Commander/Commander/Arm/MC_Mode/Auto/Offboard/Acc_Command ==
  FMS_In : Inport
  Accel_Command : Subsystem
  Body_Frame : Subsystem
  Bus Selector1 : BusSelector  OutputSignals=INS_Out.psi
  Bus Selector3 : BusSelector  OutputSignals=Auto_Cmd.frame
  Command_Mask : Subsystem
  Demux : Demux  Outputs=3
  Global_Frame : Subsystem
  Index Vector : MultiPortSwitch  DataPortOrder=Zero-based contiguous  zeroidx=on
  Local_Frame : Subsystem
  Multiply : Product
  ax_C_cmd : Outport
  ay_C_cmd : Outport  Port=2
  az_C_cmd : Outport  Port=3
  wires:
  FMS_In/1 -> Bus Selector3/1, Bus Selector1/1, Accel_Command/1(FMS_In), Command_Mask/1(FMS_In)
  Bus Selector3/1 -> Index Vector/1  "<frame>"
  Command_Mask/1(acc_mask) -> Multiply/2
  Global_Frame/1(acc_cmd_C) -> Index Vector/2
  Local_Frame/1(acc_cmd_C) -> Index Vector/3
  Body_Frame/1(acc_cmd_C) -> Index Vector/4
  Multiply/1 -> Body_Frame/1(acc_cmd_B), Global_Frame/2(acc_cmd_O), Local_Frame/2(acc_cmd_R)
  Bus Selector1/1 -> Local_Frame/1(psi), Global_Frame/1(psi)  "<psi>"
  Index Vector/1 -> Demux/1
  Demux/1 -> ax_C_cmd/1
  Demux/2 -> ay_C_cmd/1
  Demux/3 -> az_C_cmd/1
  Accel_Command/1(accel_cmd) -> Multiply/1

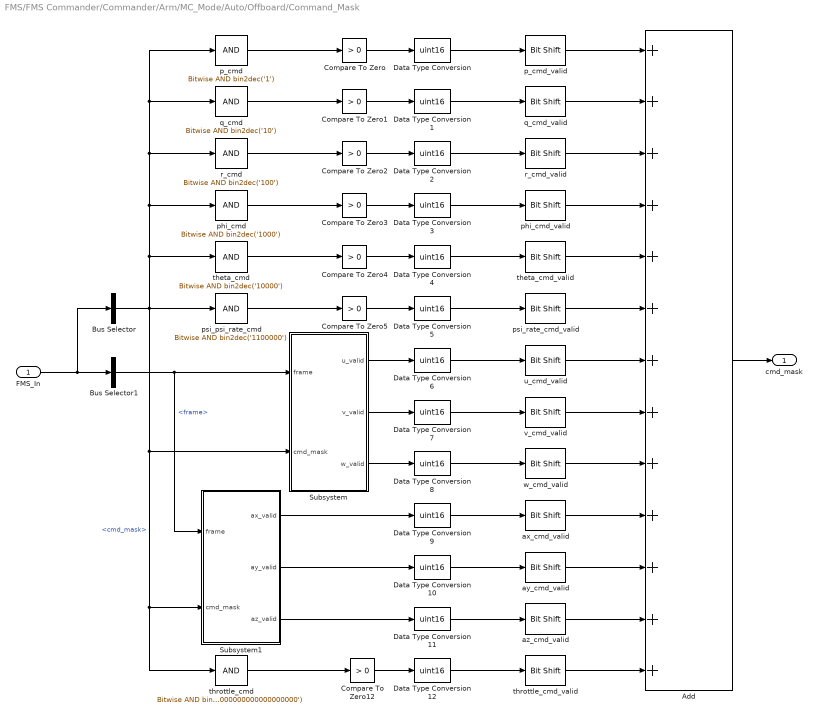
== system FMS/FMS Commander/Commander/Arm/MC_Mode/Auto/Offboard/Command_Mask ==
  FMS_In : Inport
  Add : Sum  Inputs=+++++++++++++
  Bus Selector : BusSelector  OutputSignals=Auto_Cmd.cmd_mask
  Bus Selector1 : BusSelector  OutputSignals=Auto_Cmd.frame
  Compare To Zero{,1..5,12} (7 alike) : simulink/Logic and Bit Operations/Compare To Zero  relop=>  OutDataTypeStr=boolean
  Data Type Conversion{,1..12} (13 alike) : DataTypeConversion  OutDataTypeStr=uint16
  Subsystem : Subsystem
  Subsystem1 : Subsystem
  ax_cmd_valid : hdlsllib/Logic and Bit Operations/Bit Shift  mode=Shift Left Logical  N=9
      settings: SourceProductName=HDL Coder  SourceProductBaseCode=HD
  ay_cmd_valid : hdlsllib/Logic and Bit Operations/Bit Shift  mode=Shift Left Logical  N=10
      settings: SourceProductName=HDL Coder  SourceProductBaseCode=HD
  az_cmd_valid : hdlsllib/Logic and Bit Operations/Bit Shift  mode=Shift Left Logical  N=11
      settings: SourceProductName=HDL Coder  SourceProductBaseCode=HD
  p_cmd : simulink/Logic and Bit Operations/Bitwise Operator  logicop=AND  UseBitMask=on  BitMask=bin2dec('1')  BitMaskRealWorld=Stored Integer
  p_cmd_valid : hdlsllib/Logic and Bit Operations/Bit Shift  mode=Shift Left Logical  N=0
      settings: SourceProductName=HDL Coder  SourceProductBaseCode=HD
  phi_cmd : simulink/Logic and Bit Operations/Bitwise Operator  logicop=AND  UseBitMask=on  BitMask=bin2dec('1000')  BitMaskRealWorld=Stored Integer
  phi_cmd_valid : hdlsllib/Logic and Bit Operations/Bit Shift  mode=Shift Left Logical  N=3
      settings: SourceProductName=HDL Coder  SourceProductBaseCode=HD
  psi_psi_rate_cmd : simulink/Logic and Bit Operations/Bitwise Operator  logicop=AND  UseBitMask=on  BitMask=bin2dec('1100000')  BitMaskRealWorld=Stored Integer
  psi_rate_cmd_valid : hdlsllib/Logic and Bit Operations/Bit Shift  mode=Shift Left Logical  N=5
      settings: SourceProductName=HDL Coder  SourceProductBaseCode=HD
  q_cmd : simulink/Logic and Bit Operations/Bitwise Operator  logicop=AND  UseBitMask=on  BitMask=bin2dec('10')  BitMaskRealWorld=Stored Integer
  q_cmd_valid : hdlsllib/Logic and Bit Operations/Bit Shift  mode=Shift Left Logical  N=1
      settings: SourceProductName=HDL Coder  SourceProductBaseCode=HD
  r_cmd : simulink/Logic and Bit Operations/Bitwise Operator  logicop=AND  UseBitMask=on  BitMask=bin2dec('100')  BitMaskRealWorld=Stored Integer
  r_cmd_valid : hdlsllib/Logic and Bit Operations/Bit Shift  mode=Shift Left Logical  N=2
      settings: SourceProductName=HDL Coder  SourceProductBaseCode=HD
  theta_cmd : simulink/Logic and Bit Operations/Bitwise Operator  logicop=AND  UseBitMask=on  BitMask=bin2dec('10000')  BitMaskRealWorld=Stored Integer
  theta_cmd_valid : hdlsllib/Logic and Bit Operations/Bit Shift  mode=Shift Left Logical  N=4
      settings: SourceProductName=HDL Coder  SourceProductBaseCode=HD
  throttle_cmd : simulink/Logic and Bit Operations/Bitwise Operator  logicop=AND  UseBitMask=on  BitMask=bin2dec('10000000000000000000')  BitMaskRealWorld=Stored Integer
  throttle_cmd_valid : hdlsllib/Logic and Bit Operations/Bit Shift  mode=Shift Left Logical  N=12
      settings: SourceProductName=HDL Coder  SourceProductBaseCode=HD
  u_cmd_valid : hdlsllib/Logic and Bit Operations/Bit Shift  mode=Shift Left Logical  N=6
      settings: SourceProductName=HDL Coder  SourceProductBaseCode=HD
  v_cmd_valid : hdlsllib/Logic and Bit Operations/Bit Shift  mode=Shift Left Logical  N=7
      settings: SourceProductName=HDL Coder  SourceProductBaseCode=HD
  w_cmd_valid : hdlsllib/Logic and Bit Operations/Bit Shift  mode=Shift Left Logical  N=8
      settings: SourceProductName=HDL Coder  SourceProductBaseCode=HD
  cmd_mask : Outport
  wires:
  FMS_In/1 -> Bus Selector/1, Bus Selector1/1
  p_cmd/1 -> Compare To Zero/1
  Compare To Zero/1 -> Data Type Conversion/1
  Data Type Conversion/1 -> p_cmd_valid/1
  q_cmd/1 -> Compare To Zero1/1
  Compare To Zero1/1 -> Data Type Conversion1/1
  Data Type Conversion1/1 -> q_cmd_valid/1
  r_cmd/1 -> Compare To Zero2/1
  Compare To Zero2/1 -> Data Type Conversion2/1
  Data Type Conversion2/1 -> r_cmd_valid/1
  Data Type Conversion3/1 -> phi_cmd_valid/1
  phi_cmd/1 -> Compare To Zero3/1
  Compare To Zero3/1 -> Data Type Conversion3/1
  Data Type Conversion4/1 -> theta_cmd_valid/1
  theta_cmd/1 -> Compare To Zero4/1
  Compare To Zero4/1 -> Data Type Conversion4/1
  psi_psi_rate_cmd/1 -> Compare To Zero5/1
  Compare To Zero5/1 -> Data Type Conversion5/1
  Data Type Conversion5/1 -> psi_rate_cmd_valid/1
  Data Type Conversion9/1 -> ax_cmd_valid/1
  Bus Selector/1 -> q_cmd/1, p_cmd/1, r_cmd/1, phi_cmd/1, theta_cmd/1, throttle_cmd/1, Subsystem1/2(cmd_mask), Subsystem/2(cmd_mask), psi_psi_rate_cmd/1  "<cmd_mask>"
  Data Type Conversion10/1 -> ay_cmd_valid/1
  Data Type Conversion11/1 -> az_cmd_valid/1
  throttle_cmd/1 -> Compare To Zero12/1
  Compare To Zero12/1 -> Data Type Conversion12/1
  Data Type Conversion12/1 -> throttle_cmd_valid/1
  p_cmd_valid/1 -> Add/1
  q_cmd_valid/1 -> Add/2
  r_cmd_valid/1 -> Add/3
  phi_cmd_valid/1 -> Add/4
  theta_cmd_valid/1 -> Add/5
  psi_rate_cmd_valid/1 -> Add/6
  ax_cmd_valid/1 -> Add/10
  ay_cmd_valid/1 -> Add/11
  az_cmd_valid/1 -> Add/12
  throttle_cmd_valid/1 -> Add/13
  Add/1 -> cmd_mask/1
  u_cmd_valid/1 -> Add/7
  v_cmd_valid/1 -> Add/8
  w_cmd_valid/1 -> Add/9
  Data Type Conversion7/1 -> v_cmd_valid/1
  Data Type Conversion8/1 -> w_cmd_valid/1
  Data Type Conversion6/1 -> u_cmd_valid/1
  Subsystem/1(u_valid) -> Data Type Conversion6/1
  Subsystem/2(v_valid) -> Data Type Conversion7/1
  Subsystem/3(w_valid) -> Data Type Conversion8/1
  Bus Selector1/1 -> Subsystem/1(frame), Subsystem1/1(frame)  "<frame>"
  Subsystem1/1(ax_valid) -> Data Type Conversion9/1
  Subsystem1/2(ay_valid) -> Data Type Conversion10/1
  Subsystem1/3(az_valid) -> Data Type Conversion11/1

== system FMS/FMS Commander/Commander/Arm/MC_Mode/Auto/Offboard/Heading_Command ==
  FMS_In : Inport
  Heading_Control : Subsystem
  Psi_Rate_Command : Subsystem
  Saturation : Saturate  UpperLimit=FMS_PARAM.YAW_RATE_LIM  LowerLimit=-FMS_PARAM.YAW_RATE_LIM
  Sum : Sum  Inputs=|++
  psi_rate_cmd : Outport
  wires:
  Sum/1 -> Saturation/1
  FMS_In/1 -> Heading_Control/1(FMS_In), Psi_Rate_Command/1(FMS_In)
  Heading_Control/1(psi_rate_cmd) -> Sum/1
  Psi_Rate_Command/1(psi_rate_cmd) -> Sum/2
  Saturation/1 -> psi_rate_cmd/1

== system FMS/FMS Commander/Commander/Arm/MC_Mode/Auto/Offboard/Velocity_Command ==
  FMS_In : Inport
  Demux : Demux  Outputs=3
  Position_Control : Subsystem
  Saturation1 : Saturate  UpperLimit=FMS_PARAM.VEL_XY_LIM  LowerLimit=-FMS_PARAM.VEL_XY_LIM
  Saturation2 : Saturate  UpperLimit=FMS_PARAM.VEL_XY_LIM  LowerLimit=-FMS_PARAM.VEL_XY_LIM
  Saturation3 : Saturate  UpperLimit=FMS_PARAM.VEL_Z_LIM  LowerLimit=-FMS_PARAM.VEL_Z_LIM
  Sum1 : Sum  Inputs=|++
  Velocity_Command : Subsystem
  u_cmd : Outport
  v_cmd : Outport  Port=2
  w_cmd : Outport  Port=3
  wires:
  FMS_In/1 -> Velocity_Command/1(FMS_In), Position_Control/1(FMS_In)
  Position_Control/1(vel_cmd_C) -> Sum1/1
  Velocity_Command/1(vel_cmd_C) -> Sum1/2
  Demux/1 -> Saturation2/1
  Demux/2 -> Saturation1/1
  Demux/3 -> Saturation3/1
  Sum1/1 -> Demux/1
  Saturation2/1 -> u_cmd/1
  Saturation1/1 -> v_cmd/1
  Saturation3/1 -> w_cmd/1

== system FMS/FMS Commander/Commander/Arm/MC_Mode/SubMode/Hold/Altitude Hold ==
  FMS_In : Inport
  Controller : Subsystem
  Detect Movement : Subsystem
  w_cmd_mPs : Outport
  wires:
  Controller/1(w_cmd_mPs) -> w_cmd_mPs/1
  Detect Movement/1(motion_state) -> Controller/1(motion_state)
  FMS_In/1 -> Controller/2(FMS_In), Detect Movement/1(FMS_In)

== system FMS/FMS Commander/Commander/Arm/MC_Mode/SubMode/Hold/Heading Hold ==
  FMS_In : Inport
  Bus Selector : BusSelector  OutputSignals=Cmd_In.set_yaw
  Compare To Zero : simulink/Logic and Bit Operations/Compare To Zero  relop=<  OutDataTypeStr=boolean
  Controller : Subsystem
  Detect Movement : Subsystem
  Heading Control : Subsystem
  Switch : Switch
  psi_rate_cmd_radPs : Outport
  wires:
  Controller/1(psi_rate_cmd_radPs) -> Switch/3
  Detect Movement/1(motion_state) -> Controller/1(motion_state)
  FMS_In/1 -> Heading Control/1(FMS_In), Bus Selector/1, Detect Movement/1(FMS_In), Controller/2(FMS_In)
  Heading Control/1(psi_rate_cmd_radPs) -> Switch/1
  Switch/1 -> psi_rate_cmd_radPs/1
  Bus Selector/1 -> Compare To Zero/1, Switch/2  "<set_yaw>"
  Compare To Zero/1 -> Heading Control/2(reset)

== system FMS/FMS Commander/Commander/Arm/MC_Mode/SubMode/Hold/Position Hold ==
  FMS_In : Inport
  Controller : Subsystem
  Demux : Demux  Outputs=2
  Detect Movement : Subsystem
  u_cmd_mPs : Outport
  v_cmd_mPs : Outport  Port=2
  wires:
  FMS_In/1 -> Controller/2(FMS_In), Detect Movement/1(FMS_In)
  Demux/2 -> v_cmd_mPs/1
  Demux/1 -> u_cmd_mPs/1
  Controller/1(uv_cmd_mPs) -> Demux/1
  Detect Movement/1(motion_state) -> Controller/1(motion_state)

== system FMS/FMS Commander/Commander/Arm/MC_Mode/SubMode/Land/Assist Land Speed ==
  FMS_In : Inport
  Bus Selector1 : BusSelector  OutputSignals=INS_Out.flag,INS_Out.h_AGL
  Compare To Constant : simulink/Logic and Bit Operations/Compare To Constant  relop=<=  const=FMS_PARAM.ASSIST_LAND_H  OutDataTypeStr=boolean
  Gain : Gain  Gain=0.5
  Land_Speed : Constant  Value=FMS_PARAM.LAND_SPEED  OutDataTypeStr=Inherit: Inherit via back propagation
  Logical Operator : Logic  AllPortsSameDT=off  OutDataTypeStr=boolean
  Switch : Switch  Criteria=u2 > Threshold
  TD : Subsystem
  cmd_p valid : simulink/Logic and Bit Operations/Bitwise Operator  logicop=AND  UseBitMask=on  BitMask=bin2dec('100000000')  BitMaskRealWorld=Stored Integer
  w_cmd_mPs : Outport
  wires:
  Land_Speed/1 -> Switch/3, Gain/1
  Gain/1 -> Switch/1
  Compare To Constant/1 -> Logical Operator/2
  FMS_In/1 -> Bus Selector1/1
  cmd_p valid/1 -> Logical Operator/1  "h_AGL_valid"
  Bus Selector1/1 -> cmd_p valid/1  "<flag>"
  Bus Selector1/2 -> Compare To Constant/1  "<h_AGL>"
  Logical Operator/1 -> Switch/2
  Switch/1 -> TD/1(v)
  TD/1(v1) -> w_cmd_mPs/1

== system FMS/FMS Commander/Commander/Arm/MC_Mode/SubMode/Land/Position Command ==
  FMS_In : Inport
  land_xy_R : Inport  Port=2
  Demux : Demux  Outputs=2
  Position Control : Subsystem
  Saturation1 : Saturate  UpperLimit=FMS_PARAM.VEL_XY_LIM/5  LowerLimit=-FMS_PARAM.VEL_XY_LIM/5
  u_cmd_mPs : Outport
  v_cmd_mPs : Outport  Port=2
  wires:
  land_xy_R/1 -> Position Control/2(land_xy_R)
  Position Control/1(uv_cmd_mPs) -> Saturation1/1
  Demux/2 -> v_cmd_mPs/1
  Demux/1 -> u_cmd_mPs/1
  Saturation1/1 -> Demux/1
  FMS_In/1 -> Position Control/1(FMS_In)

== system FMS/FMS Commander/Commander/Arm/MC_Mode/SubMode/Return/Heading Commander ==
  FMS_In : Inport
  p1p2 : Inport  Port=2
  Heading Control : Subsystem
  Included Angle : Subsystem
  North : Constant  Value=[1 0]  OutDataTypeStr=single
  psi_err_rad : Outport
  psi_rad_cmd : Outport  Port=2
  wires:
  p1p2/1 -> Included Angle/2(vec2)
  FMS_In/1 -> Heading Control/1(FMS_In)
  North/1 -> Included Angle/1(vec1)
  Included Angle/1(angle_rad) -> Heading Control/2(psi_cmd_rad)
  Heading Control/1(psi_rate_cmd_radPs) -> psi_rad_cmd/1
  Heading Control/2(psi_err_rad) -> psi_err_rad/1

== system FMS/FMS Commander/Commander/Arm/MC_Mode/SubMode/Return/Velocity Commander ==
  p1 : Inport
  p2 : Inport  Port=2
  p3 : Inport  Port=3
  L1 : Inport  Port=4
  In Bus Element3 : Inport  Port=5  PortName=FMS_In
  In Bus Element : Inport  Port=5  PortName=FMS_In  Element=INS_Out.vn
  In Bus Element1 : Inport  Port=5  PortName=FMS_In  Element=INS_Out.ve
  In Bus Element2 : Inport  Port=5  PortName=FMS_In  Element=INS_Out.psi
  psi_err_rad : Inport  Port=6
  Abs : Abs
  Compare To Constant : simulink/Logic and Bit Operations/Compare To Constant  relop=<=  const=10/180*pi  OutDataTypeStr=boolean
  Compare To Zero : simulink/Logic and Bit Operations/Compare To Zero  relop===  OutDataTypeStr=boolean
  "Cruise Speed " : Subsystem
  Demux : Demux  Outputs=3
  Hold Position : Subsystem
  L1 Reference WP : Subsystem
  Lateral Acceleration : Subsystem
  Lateral Acceleration To Speed : Subsystem
  Mux1 : Mux  Inputs=2
  Switch : Switch  Criteria=u2 > Threshold
  ValidCounter : Subsystem
  u_cmd : Outport
  v_cmd : Outport  Port=2
  w_cmd : Outport  Port=3
  wires:
  p3/1 -> "Cruise Speed "/1(P3), Lateral Acceleration To Speed/2(p3), Lateral Acceleration/3(p3), L1 Reference WP/3(P3)
  In Bus Element1/1 -> Mux1/2
  Mux1/1 -> Lateral Acceleration/1(Vg)
  p2/1 -> "Cruise Speed "/2(P2), Lateral Acceleration To Speed/3(p2), L1 Reference WP/2(P2)
  Demux/2 -> v_cmd/1
  Demux/3 -> w_cmd/1
  Demux/1 -> u_cmd/1
  In Bus Element/1 -> Mux1/1
  L1 Reference WP/1(L1_WP) -> Lateral Acceleration/2(L1_WP)  "L1_WP"
  p1/1 -> L1 Reference WP/1(P1)
  L1/1 -> Lateral Acceleration/4(L1), L1 Reference WP/4(L1)
  Lateral Acceleration/1(l1_a_cmd) -> Lateral Acceleration To Speed/1(l1_a)
  In Bus Element2/1 -> Lateral Acceleration To Speed/6(psi)
  "Cruise Speed "/1(|Vg|) -> Lateral Acceleration To Speed/4(Vg)
  Lateral Acceleration To Speed/1(Vg_C_cmd) -> Switch/3
  psi_err_rad/1 -> Abs/1
  Abs/1 -> Compare To Constant/1
  In Bus Element3/1 -> Hold Position/1(FMS_In)
  Hold Position/1(vel_cmd) -> Switch/1
  Switch/1 -> Demux/1
  ValidCounter/1(out) -> Compare To Zero/1
  Compare To Constant/1 -> ValidCounter/1(in)
  Compare To Zero/1 -> Lateral Acceleration To Speed/7(rotating), "Cruise Speed "/3(rotating), Switch/2
  "Cruise Speed "/2(cruise_speed) -> Lateral Acceleration To Speed/5(cruise_speed)

== system FMS/FMS Commander/Commander/Arm/MC_Mode/SubMode/Return/Way Points ==
  note: P1: path start point
      | P2: path end point
      | P3: vehicle point
  FMS_In : Inport
  Bus Selector : BusSelector  OutputSignals=INS_Out.x_R,INS_Out.y_R
  Bus Selector1 : BusSelector  OutputSignals=Cmd_In.sp_waypoint
  Bus Selector2 : BusSelector  OutputSignals=Cmd_In.cur_waypoint
  Mux : Mux  Inputs=2
  Reshape : Reshape  OutputDimensionality=Customize  OutputDimensions=[2,1]
  Reshape1 : Reshape  OutputDimensionality=Customize  OutputDimensions=[2,1]
  Reshape2 : Reshape  OutputDimensionality=Customize  OutputDimensions=[2,1]
  Selector : Selector  InputPortWidth=3  IndexOptions=Index vector (dialog)  Indices=[1 2]  OutputSizes=1
  Selector1 : Selector  InputPortWidth=3  IndexOptions=Index vector (dialog)  Indices=[1 2]  OutputSizes=1
  p1 : Outport
  p2 : Outport  Port=2
  p3 : Outport  Port=3
  wires:
  Reshape2/1 -> p3/1
  Reshape1/1 -> p1/1
  Reshape/1 -> p2/1
  Bus Selector/2 -> Mux/2  "<y_R>"
  Bus Selector/1 -> Mux/1  "<x_R>"
  Mux/1 -> Reshape2/1
  Bus Selector1/1 -> Selector/1  "<sp_waypoint>"
  Selector/1 -> Reshape/1
  Bus Selector2/1 -> Selector1/1  "<cur_waypoint>"
  FMS_In/1 -> Bus Selector2/1, Bus Selector1/1, Bus Selector/1
  Selector1/1 -> Reshape1/1
